simulink model "L150_Closed_Loop2"  (R2026a)
settings: Solver=VariableStepAuto  StopTime=100
undefined symbols (not defined in the file): initialRoute
libraries: robotmobilelib x1, simulink x1
settings Model: Creator=hanjiatong  LastModifiedBy=hanjiatong

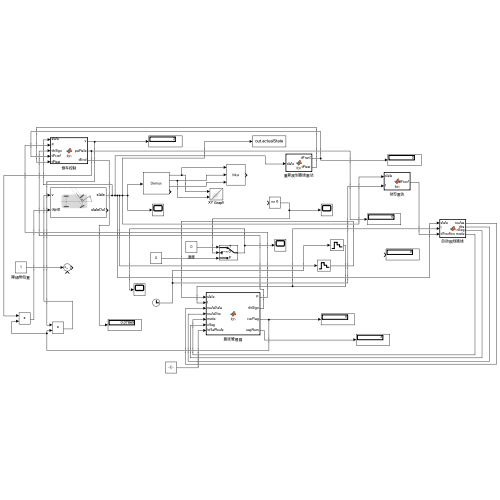
[thumbnail: Simulink's stored preview of the top-level diagram]
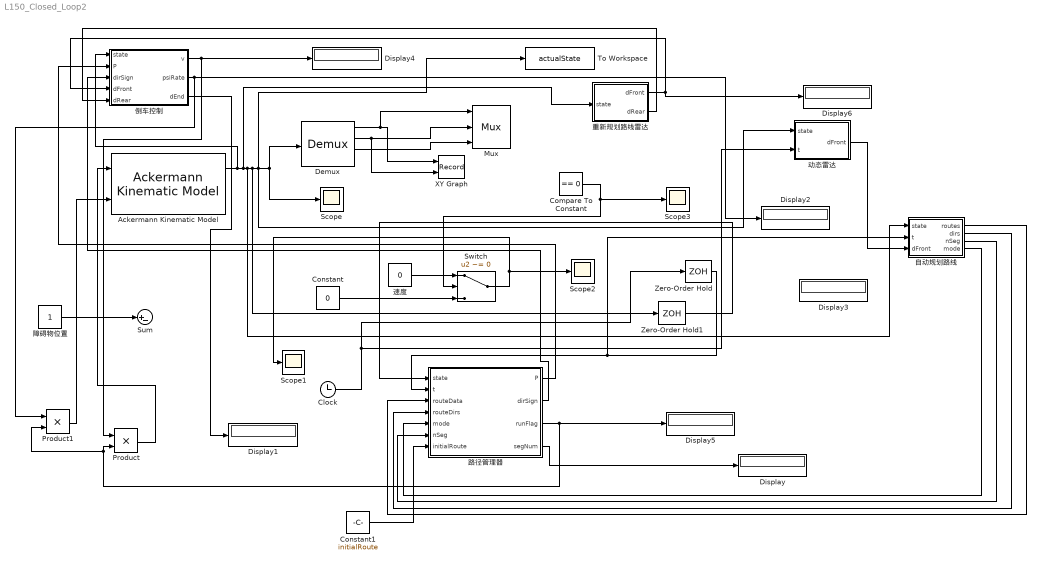
== system L150_Closed_Loop2 ==
  Ackermann Kinematic Model : robotmobilelib/Ackermann Kinematic Model  WheelBase=0.144  VehicleSpeedRange=[-inf inf]  MaxSteeringAngle=0.25  InitialState=[1;3;0;0]  SimulateUsing=Interpreted execution
  Clock : Clock
  Compare To Constant : simulink/Logic and Bit Operations/Compare To Constant  relop===  const=0  OutDataTypeStr=boolean
  Constant : Constant  Value=0
  Constant1 : Constant  Value=initialRoute
  Demux : Demux
      settings: DisplayOption=none
  Display{,1..6} (7 alike) : Display
  Mux : Mux  Inputs=3
  Product : Product
  Product1 : Product
  Scope{,1..3} (4 alike) : Scope
      Scope settings: ActiveDisplayYMinimum=-0.19594221664657985  ActiveDisplayYMaximum=1.7514452129987257
      Scope1 settings: ActiveDisplayYMinimum=-1  ActiveDisplayYMaximum=1
      Scope2 settings: ActiveDisplayYMinimum=-0.018749999999999996  ActiveDisplayYMaximum=0.16874999999999998  DataLoggingVariableName=ScopeData2
      Scope3 settings: ActiveDisplayYMinimum=0.33124999999999571  ActiveDisplayYMaximum=1.018749999999998  DataLoggingVariableName=ScopeData3
  Sum : Sum  Inputs=|+-
  Switch : Switch  Criteria=u2 ~= 0  SaturateOnIntegerOverflow=off  InputSameDT=off
  To Workspace : ToWorkspace  VariableName=actualState  SaveFormat=Timeseries  SampleTime=-1
  XY Graph : Record  NumPorts=2.0  FileSettingsInternal="{\"entries\":[{\"content\":{\"excelSettings\":{\"content\":{},\"type\":\"Streamout.ExcelSettings\"},\"parquetSettings\":{\"content\":{},\"type\":\"Streamout.ParquetSettings\"}},\"type\":\"Streamout.FileSettingStorage\",\"uuid\":\"\"}],\"packageUris\":[\"http:\\/\\/schema.mathworks.com\\/mf0\\/streamout_blocks\\/R2020a\"],\"version\":\"1.0\"}"  FrameSettings=[0, 0]  Layout=[1 1]  SignalsInternal="{\"entries\":[{\"content\":{\"signals\":[{\"content\":{\"blockPath\":[],\"dimensions\":[1],\"domain\":\"\",\"lineColor\":\"#a2142f\",\"plots\":[ 1 ],\"port\":1,\"sid\":[\"\"],\"signalID\":1,\"signalName\":\"Demux:1\"},\"type\":\"RecordBlkView.Signal\",\"uuid\":\"\"},{\"content\":{\"blockPath\":[],\"dimensions\":[1],\"domain\":\"\",\"lineColor\":\"#139fff\",\"plots\":[ 1 ],\"port\":2,\"sid\":[\"\"],\"signalID\":2,\"signalName\":\"Demux:2\"},\"type\":\"RecordBlkView.Signal\",\"uuid\":\"\"}]},\"type\":\"RecordBlkView.InputSignals\",\"uuid\":\"\"}],\"packageUris\":[\"http:\\/\\/schema.mathworks.com\\/mf0\\/streamout_blocks\\/R2020a\"],\"version\":\"1.0\"}"  VisualizationBindings="{\"xyplotplugin\":{\"info\":[{\"series\":[{\"bindingParametersList\":[{\"parameter\":\"X-Axis\",\"signalID\":1,\"signalName\":\"Demux:1\"},{\"parameter\":\"Y-Axis\",\"signalID\":2,\"signalName\":\"Demux:2\"}],\"seriesID\":0}],\"subplotID\":1}]}}"  CompatibilityTag=XY
  Zero-Order Hold : ZeroOrderHold  SampleTime=0.05
  Zero-Order Hold1 : ZeroOrderHold  SampleTime=0.05
  倒车控制 : MATLAB Function  TreatAsAtomicUnit=on
  动态雷达 : MATLAB Function  TreatAsAtomicUnit=on
  自动规划路线 : MATLAB Function  TreatAsAtomicUnit=on
  路径管理器 : MATLAB Function  TreatAsAtomicUnit=on
  速度 : Constant  Value=0
  重新规划路线雷达 : MATLAB Function  TreatAsAtomicUnit=on
  障碍物位置 : Constant
  wires:
  Ackermann Kinematic Model/1 -> 倒车控制/1(state), 重新规划路线雷达/1(state), 自动规划路线/1(state), Zero-Order Hold1/1, 动态雷达/1(state), Scope/1, Demux/1, To Workspace/1
  Demux/2 -> XY Graph/2, Mux/2
  障碍物位置/1 -> Sum/1
  Switch/1 -> Scope2/1, Scope1/1
  Compare To Constant/1 -> Scope3/1, Switch/2
  速度/1 -> Switch/1
  Constant/1 -> Switch/3
  Demux/1 -> Mux/1, XY Graph/1
  Demux/3 -> Mux/3
  重新规划路线雷达/1(dFront) -> 倒车控制/4(dFront), Display6/1
  重新规划路线雷达/2(dRear) -> 倒车控制/5(dRear)
  倒车控制/1(v) -> Product/1, Display4/1
  倒车控制/2(psiRate) -> Product1/1, Display2/1
  倒车控制/3(dEnd) -> Display1/1
  Clock/1 -> 动态雷达/2(t), Zero-Order Hold/1
  自动规划路线/1(routes) -> 路径管理器/3(routeData)
  路径管理器/1(P) -> 倒车控制/2(P)
  路径管理器/2(dirSign) -> 倒车控制/3(dirSign)
  自动规划路线/2(dirs) -> 路径管理器/4(routeDirs)
  Zero-Order Hold/1 -> 自动规划路线/2(t), 路径管理器/2(t)
  Zero-Order Hold1/1 -> 路径管理器/1(state)
  路径管理器/3(runFlag) -> Product1/2, Product/2, Display5/1
  Product/1 -> Ackermann Kinematic Model/1
  Product1/1 -> Ackermann Kinematic Model/2
  路径管理器/4(segNum) -> Display/1
  动态雷达/1(dFront) -> 自动规划路线/3(dFront)
  自动规划路线/4(mode) -> 路径管理器/5(mode)
  自动规划路线/3(nSeg) -> 路径管理器/6(nSeg)
  Constant1/1 -> 路径管理器/7(initialRoute)

== matlab function L150_Closed_Loop2/自动规划路线 ==
  settings: updateMethod=DISCRETE  sampleTime=0.05
  data: state input; routes output; t input; dFront input; dirs output; nSeg output; mode output

function [routes,dirs,nSeg,mode] = fcn(state,t,dFront)

% mode:
% 0 = 沿原路线行驶
% 1 = 停车并准备切换
% 2 = 执行新路线
% 3 = 规划失败，保持停车

coder.extrinsic('l150AutoReplan');

persistent savedRoutes savedDirs savedN ...
           phase stopTime lastT

if isempty(phase)
    savedRoutes = zeros(256,2,10);
    savedDirs = zeros(10,1);
    savedN = 0;
    phase = 0;
    stopTime = 0;
    lastT = -1;
end

% 仿真重新开始时复位
if t < lastT - 1e-6
    savedRoutes = zeros(256,2,10);
    savedDirs = zeros(10,1);
    savedN = 0;
    phase = 0;
    stopTime = 0;
end
lastT = t;

% 测试用：新障碍物在第15秒出现后立即重新规划
if phase == 0 && t >= 15
    % 预先定义输出类型和尺寸
    newRoutes = zeros(256,2,10);
    newDirs = zeros(10,1);
    newN = 0;
    ok = 0;

    % 调用之前写好的 Hybrid A* 函数
    [newRoutes,newDirs,newN,ok] = ...
        l150AutoReplan(state(1:3));

    if ok == 1 && newN > 0
        savedRoutes = newRoutes;
        savedDirs = newDirs;
        savedN = newN;

        phase = 1;
        stopTime = t;
    else
        phase = 3;
    end
end

% 停车0.6秒，再执行新路线
if phase == 1 && t-stopTime >= 0.6
    phase = 2;
end

routes = savedRoutes;
dirs = savedDirs;
nSeg = savedN;
mode = phase;

end

== matlab function L150_Closed_Loop2/路径管理器 ==
  data: state input; P output; t input; routeData input; routeDirs input; dirSign output; runFlag output; segNum output; mode input; nSeg input; initialRoute input

function [P,dirSign,runFlag,segNum] = ...
    fcn(state,t,routeData,routeDirs,mode,nSeg,initialRoute)

% mode=0：执行原路线
% mode=1：停车，等待重新规划路线切换
% mode=2：执行新路线
% mode=3：规划失败，停车

persistent k phase holdTime previousMode previousT

if isempty(k)
    k = 1;
    phase = 0;
    holdTime = 0;
    previousMode = -1;
    previousT = -1;
end

% 重新运行仿真时复位
if t < previousT - 1e-6
    k = 1;
    phase = 0;
    holdTime = 0;
    previousMode = -1;
end

% 第一次进入新路线模式
if mode == 2 && previousMode ~= 2
    k = 1;
    phase = 0;
    holdTime = t;
end

previousMode = mode;
previousT = t;

% 默认保持停车
P = initialRoute;
dirSign = 1;
runFlag = 0;
segNum = 0;

% 沿最初的规划路线行驶
if mode == 0
    runFlag = 1;
    return;
end

% 停车等待或规划失败
if mode ~= 2
    return;
end

% 自动重规划返回的有效路段数
N = min(max(floor(nSeg),0), ...
        size(routeData,3));

if N < 1
    return;
end

k = min(max(k,1),N);

% 当前路段
P = routeData(:,:,k);

% 距离路段终点
dEnd = hypot(P(end,1)-state(1), ...
             P(end,2)-state(2));

% 行驶过程中到达路段终点
if phase == 0 && dEnd <= 0.08

    if k == N
        phase = 2;  % 全部完成
    else
        phase = 1;  % 开始停车换挡
        holdTime = t;
    end

% 换挡等待0.6秒
elseif phase == 1 && t-holdTime >= 0.6
    k = k + 1;
    phase = 0;
end

% 更新当前路线
P = routeData(:,:,k);
dirSign = routeDirs(k);
segNum = k;

dEnd = hypot(P(end,1)-state(1), ...
             P(end,2)-state(2));

runFlag = double(phase == 0 && dEnd > 0.08);

end

== matlab function L150_Closed_Loop2/动态雷达 ==
  data: state input; dFront output; t input

function dFront = fcn(state,t)

coder.extrinsic('l150DynamicFront');

% 小车当前位置和朝向
pose = [state(1),state(2),state(3)];

% 初始化输出
dFront = 3.0;

% 调用之前写好的动态雷达函数
dFront = l150DynamicFront(pose,t);

end

== matlab function L150_Closed_Loop2/重新规划路线雷达 ==
  data: state input; dFront output; dRear output

function [dFront,dRear] = fcn(state)

coder.extrinsic('l150ReplanLidar');

pose = [state(1),state(2),state(3)];

dFront = 3.0;
dRear = 3.0;

[dFront,dRear] = l150ReplanLidar(pose);

end

== matlab function L150_Closed_Loop2/倒车控制 ==
  data: state input; v output; P input; dirSign input; dFront input; dRear input; psiRate output; dEnd output

function [v,psiRate,dEnd] = fcn( ...
    state,P,dirSign,dFront,dRear)

% state = [x y theta psi]
% P：当前要跟踪的一段路径
% dirSign：1前进，-1倒车

x = state(1);
y = state(2);
theta = state(3);
psi = state(4);

v = 0;
psiRate = 0;

% 当前路段终点距离
dEnd = hypot(P(end,1)-x,P(end,2)-y);

% 到达路段终点，停车
if dEnd <= 0.08
    return;
end

% 按行驶方向选择速度和安全雷达

% 仿真测试：按照规划方向行驶
% 暂时不使用雷达距离触发停车

if dirSign > 0
    v = 0.08;
else
    v = -0.06;
end


% 找出当前路段最近的路径点
n = size(P,1);
nearest = 1;
best = inf;

for i = 1:n
    d2 = (P(i,1)-x)^2 + (P(i,2)-y)^2;
    if d2 < best
        best = d2;
        nearest = i;
    end
end

% 沿路径向前寻找约0.25米的目标点
target = nearest;
travel = 0;

for i = nearest:n-1
    travel = travel + hypot( ...
        P(i+1,1)-P(i,1), ...
        P(i+1,2)-P(i,2));

    target = i+1;

    if travel >= 0.15
    break;
end
    
end

dx = P(target,1)-x;
dy = P(target,2)-y;

% 倒车时，运动方向与车头相反
moveHeading = theta;

if dirSign < 0
    moveHeading = theta + pi;
end

% 目标点在运动方向坐标系中的横向位置
yLocal = -sin(moveHeading)*dx ...
         + cos(moveHeading)*dy;

L2 = max(dx^2+dy^2,0.12^2);

% Pure Pursuit 几何曲率
kappa = 2*yLocal/L2;

% 倒车时需要反转转向曲率的符号
psiTarget = atan(0.144*dirSign*kappa);

% 限制转向角
psiTarget = max(-0.25,min(0.25,psiTarget));

% 计算前轮转向角速度
psiRate = 2*(psiTarget-psi);

% 限制转向角速度
psiRate = max(-0.35,min(0.35,psiRate));

end
